simulink model "fault_detection_system_v3_updated"  (R2024a)
settings: Solver=FixedStepDiscrete  StartTime=0.0  StopTime=2.2  FixedStep=1e-4  RelTol=1e-3
settings Model: Creator=UJJWAL  LastModifiedBy=UJJWAL

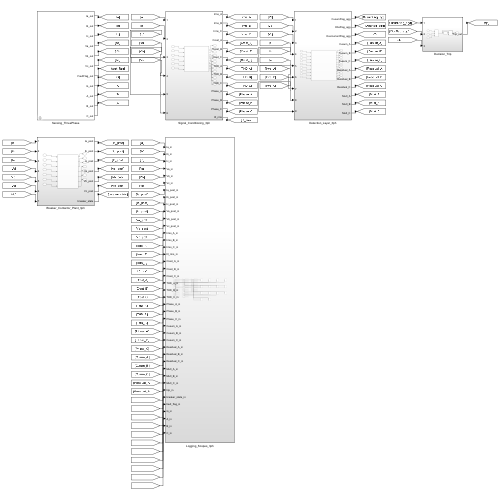
[thumbnail: Simulink's stored preview of the top-level diagram]
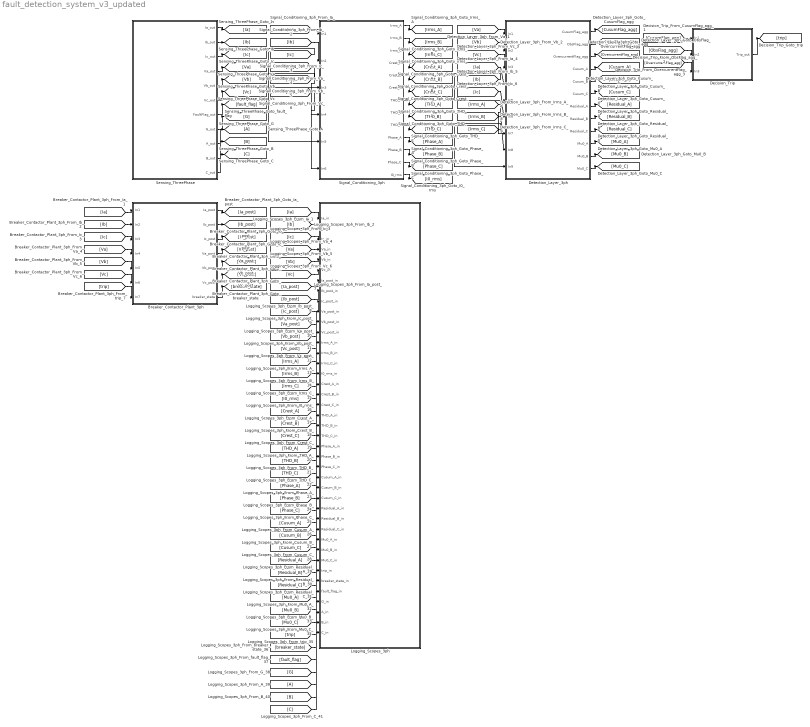
== system fault_detection_system_v3_updated ==
  Breaker_Contactor_Plant_3ph : Subsystem
  Decision_Trip : Subsystem
  Detection_Layer_3ph : Subsystem
  Logging_Scopes_3ph : Subsystem
  Logging_Scopes_3ph_From_A_39 : From
  Sensing_ThreePhase : Subsystem  mask{FaultG=off, FaultA=on, FaultB=on, FaultC=on, MechanismCode=6, Severity=1790.2024, RampDuration=0, FaultOnsetTime=0.7, FaultDuration=1, NoiseSeed=2700, NoiseI=0.3, NoiseV=3}
      mask prompts: FaultG "Ground involved (G)"; FaultA "Phase A involved"; FaultB "Phase B involved"; FaultC "Phase C involved"; MechanismCode "Mechanism code (1=Healthy, 2=ShortCircuit, 3=Overcurrent, 4=Overvoltage, 5=Undervoltage, 6=OpenCircuit)"; RampDuration "Ramp duration (s)"; FaultOnsetTime "Fault onset time (s)"; FaultDuration "Fault duration (s)"; NoiseSeed "Noise seed"; NoiseI "Current sensor noise (A, per sample)"; NoiseV "Voltage sensor noise (V, per sample)"
  Sensing_ThreePhase_Goto_A : Goto
  Signal_Conditioning_3ph : Subsystem
  wires:
  Sensing_ThreePhase/1(Ia_out) -> [Ia]
  Sensing_ThreePhase/2(Ib_out) -> [Ib]
  Sensing_ThreePhase/3(Ic_out) -> [Ic]
  Sensing_ThreePhase/4(Va_out) -> [Va]
  Sensing_ThreePhase/5(Vb_out) -> [Vb]
  Sensing_ThreePhase/6(Vc_out) -> [Vc]
  Sensing_ThreePhase/7(FaultFlag_out) -> [fault_flag]
  Sensing_ThreePhase/8(G_out) -> [G]
  Sensing_ThreePhase/9(A_out) -> Sensing_ThreePhase_Goto_A/1
  Sensing_ThreePhase/10(B_out) -> [B]
  Sensing_ThreePhase/11(C_out) -> [C]
  Signal_Conditioning_3ph/1(Irms_A) -> [Irms_A]
  Signal_Conditioning_3ph/2(Irms_B) -> [Irms_B]
  Signal_Conditioning_3ph/3(Irms_C) -> [Irms_C]
  Signal_Conditioning_3ph/4(Crest_A) -> [Crest_A]
  Signal_Conditioning_3ph/5(Crest_B) -> [Crest_B]
  Signal_Conditioning_3ph/6(Crest_C) -> [Crest_C]
  Signal_Conditioning_3ph/7(THD_A) -> [THD_A]
  Signal_Conditioning_3ph/8(THD_B) -> [THD_B]
  Signal_Conditioning_3ph/9(THD_C) -> [THD_C]
  Signal_Conditioning_3ph/10(Phase_A) -> [Phase_A]
  Signal_Conditioning_3ph/11(Phase_B) -> [Phase_B]
  Signal_Conditioning_3ph/12(Phase_C) -> [Phase_C]
  Signal_Conditioning_3ph/13(I0_rms) -> [I0_rms]
  Detection_Layer_3ph/1(CusumFlag_agg) -> [CusumFlag_agg]
  Detection_Layer_3ph/2(ObsFlag_agg) -> [ObsFlag_agg]
  Detection_Layer_3ph/3(OvercurrentFlag_agg) -> [OvercurrentFlag_agg]
  Detection_Layer_3ph/4(Cusum_A) -> [Cusum_A]
  Detection_Layer_3ph/5(Cusum_B) -> [Cusum_B]
  Detection_Layer_3ph/6(Cusum_C) -> [Cusum_C]
  Detection_Layer_3ph/7(Residual_A) -> [Residual_A]
  Detection_Layer_3ph/8(Residual_B) -> [Residual_B]
  Detection_Layer_3ph/9(Residual_C) -> [Residual_C]
  Detection_Layer_3ph/10(Mu0_A) -> [Mu0_A]
  Detection_Layer_3ph/11(Mu0_B) -> [Mu0_B]
  Detection_Layer_3ph/12(Mu0_C) -> [Mu0_C]
  Decision_Trip/1(Trip_out) -> [trip]
  Breaker_Contactor_Plant_3ph/1(Ia_post) -> [Ia_post]
  Breaker_Contactor_Plant_3ph/2(Ib_post) -> [Ib_post]
  Breaker_Contactor_Plant_3ph/3(Ic_post) -> [Ic_post]
  Breaker_Contactor_Plant_3ph/4(Va_post) -> [Va_post]
  Breaker_Contactor_Plant_3ph/5(Vb_post) -> [Vb_post]
  Breaker_Contactor_Plant_3ph/6(Vc_post) -> [Vc_post]
  Breaker_Contactor_Plant_3ph/7(breaker_state) -> [breaker_state]
  [Ia] -> Signal_Conditioning_3ph/1(In1)
  [Ib] -> Signal_Conditioning_3ph/2(In2)
  [Ic] -> Signal_Conditioning_3ph/3(In3)
  [Va] -> Signal_Conditioning_3ph/4(In4)
  [Vb] -> Signal_Conditioning_3ph/5(In5)
  [Vc] -> Signal_Conditioning_3ph/6(In6)
  [Va] -> Detection_Layer_3ph/1(In1)
  [Vb] -> Detection_Layer_3ph/2(In2)
  [Vc] -> Detection_Layer_3ph/3(In3)
  [Ia] -> Detection_Layer_3ph/4(In4)
  [Ib] -> Detection_Layer_3ph/5(In5)
  [Ic] -> Detection_Layer_3ph/6(In6)
  [Irms_A] -> Detection_Layer_3ph/7(In7)
  [Irms_B] -> Detection_Layer_3ph/8(In8)
  [Irms_C] -> Detection_Layer_3ph/9(In9)
  [CusumFlag_agg] -> Decision_Trip/1(In1)
  [ObsFlag_agg] -> Decision_Trip/2(In2)
  [OvercurrentFlag_agg] -> Decision_Trip/3(In3)
  [Ia] -> Breaker_Contactor_Plant_3ph/1(In1)
  [Ib] -> Breaker_Contactor_Plant_3ph/2(In2)
  [Ic] -> Breaker_Contactor_Plant_3ph/3(In3)
  [Va] -> Breaker_Contactor_Plant_3ph/4(In4)
  [Vb] -> Breaker_Contactor_Plant_3ph/5(In5)
  [Vc] -> Breaker_Contactor_Plant_3ph/6(In6)
  [trip] -> Breaker_Contactor_Plant_3ph/7(In7)
  [Ia] -> Logging_Scopes_3ph/1(Ia_in)
  [Ib] -> Logging_Scopes_3ph/2(Ib_in)
  [Ic] -> Logging_Scopes_3ph/3(Ic_in)
  [Va] -> Logging_Scopes_3ph/4(Va_in)
  [Vb] -> Logging_Scopes_3ph/5(Vb_in)
  [Vc] -> Logging_Scopes_3ph/6(Vc_in)
  [Ia_post] -> Logging_Scopes_3ph/7(Ia_post_in)
  [Ib_post] -> Logging_Scopes_3ph/8(Ib_post_in)
  [Ic_post] -> Logging_Scopes_3ph/9(Ic_post_in)
  [Va_post] -> Logging_Scopes_3ph/10(Va_post_in)
  [Vb_post] -> Logging_Scopes_3ph/11(Vb_post_in)
  [Vc_post] -> Logging_Scopes_3ph/12(Vc_post_in)
  [Irms_A] -> Logging_Scopes_3ph/13(Irms_A_in)
  [Irms_B] -> Logging_Scopes_3ph/14(Irms_B_in)
  [Irms_C] -> Logging_Scopes_3ph/15(Irms_C_in)
  [I0_rms] -> Logging_Scopes_3ph/16(I0_rms_in)
  [Crest_A] -> Logging_Scopes_3ph/17(Crest_A_in)
  [Crest_B] -> Logging_Scopes_3ph/18(Crest_B_in)
  [Crest_C] -> Logging_Scopes_3ph/19(Crest_C_in)
  [THD_A] -> Logging_Scopes_3ph/20(THD_A_in)
  [THD_B] -> Logging_Scopes_3ph/21(THD_B_in)
  [THD_C] -> Logging_Scopes_3ph/22(THD_C_in)
  [Phase_A] -> Logging_Scopes_3ph/23(Phase_A_in)
  [Phase_B] -> Logging_Scopes_3ph/24(Phase_B_in)
  [Phase_C] -> Logging_Scopes_3ph/25(Phase_C_in)
  [Cusum_A] -> Logging_Scopes_3ph/26(Cusum_A_in)
  [Cusum_B] -> Logging_Scopes_3ph/27(Cusum_B_in)
  [Cusum_C] -> Logging_Scopes_3ph/28(Cusum_C_in)
  [Residual_A] -> Logging_Scopes_3ph/29(Residual_A_in)
  [Residual_B] -> Logging_Scopes_3ph/30(Residual_B_in)
  [Residual_C] -> Logging_Scopes_3ph/31(Residual_C_in)
  [Mu0_A] -> Logging_Scopes_3ph/32(Mu0_A_in)
  [Mu0_B] -> Logging_Scopes_3ph/33(Mu0_B_in)
  [Mu0_C] -> Logging_Scopes_3ph/34(Mu0_C_in)
  [trip] -> Logging_Scopes_3ph/35(trip_in)
  [breaker_state] -> Logging_Scopes_3ph/36(breaker_state_in)
  [fault_flag] -> Logging_Scopes_3ph/37(fault_flag_in)
  [G] -> Logging_Scopes_3ph/38(G_in)
  Logging_Scopes_3ph_From_A_39/1 -> Logging_Scopes_3ph/39(A_in)
  [B] -> Logging_Scopes_3ph/40(B_in)
  [C] -> Logging_Scopes_3ph/41(C_in)

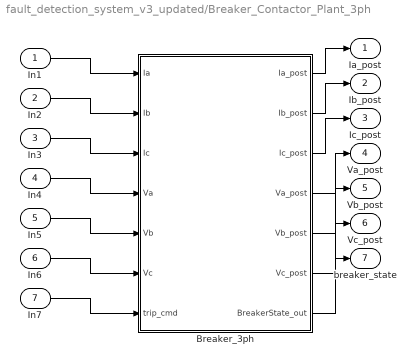
== system fault_detection_system_v3_updated/Breaker_Contactor_Plant_3ph ==
  In1 : Inport
  In2 : Inport  Port=2
  In3 : Inport  Port=3
  In4 : Inport  Port=4
  In5 : Inport  Port=5
  In6 : Inport  Port=6
  In7 : Inport  Port=7
  Breaker_3ph : MATLAB Function  TreatAsAtomicUnit=on
  Ia_post : Outport
  Ib_post : Outport  Port=2
  Ic_post : Outport  Port=3
  Va_post : Outport  Port=4
  Vb_post : Outport  Port=5
  Vc_post : Outport  Port=6
  breaker_state : Outport  Port=7
  wires:
  Breaker_3ph/1(Ia_post) -> Ia_post/1
  Breaker_3ph/2(Ib_post) -> Ib_post/1
  Breaker_3ph/3(Ic_post) -> Ic_post/1
  Breaker_3ph/4(Va_post) -> Va_post/1
  Breaker_3ph/5(Vb_post) -> Vb_post/1
  Breaker_3ph/6(Vc_post) -> Vc_post/1
  Breaker_3ph/7(BreakerState_out) -> breaker_state/1
  In1/1 -> Breaker_3ph/1(Ia)
  In2/1 -> Breaker_3ph/2(Ib)
  In3/1 -> Breaker_3ph/3(Ic)
  In4/1 -> Breaker_3ph/4(Va)
  In5/1 -> Breaker_3ph/5(Vb)
  In6/1 -> Breaker_3ph/6(Vc)
  In7/1 -> Breaker_3ph/7(trip_cmd)

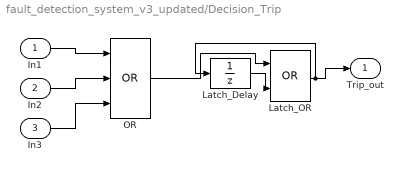
== system fault_detection_system_v3_updated/Decision_Trip ==
  In1 : Inport
  In2 : Inport  Port=2
  In3 : Inport  Port=3
  Latch_Delay : UnitDelay  SampleTime=-1  HasFrameUpgradeWarning=on
  Latch_OR : Logic  Operator=OR  AllPortsSameDT=off  OutDataTypeStr=boolean
  OR : Logic  Operator=OR  Inputs=3  AllPortsSameDT=off  OutDataTypeStr=boolean
  Trip_out : Outport
  wires:
  In1/1 -> OR/1
  In2/1 -> OR/2
  In3/1 -> OR/3
  OR/1 -> Latch_OR/1
  Latch_Delay/1 -> Latch_OR/2
  Latch_OR/1 -> Latch_Delay/1, Trip_out/1

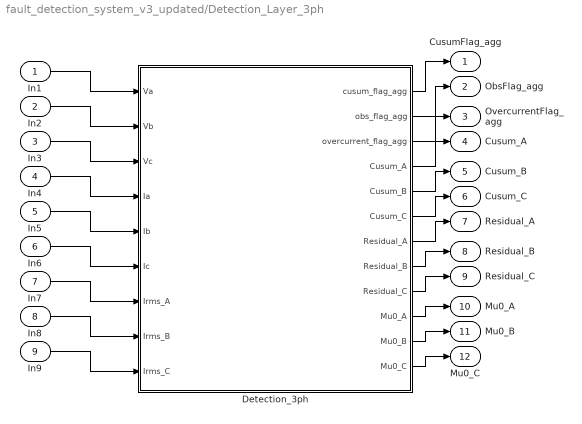
== system fault_detection_system_v3_updated/Detection_Layer_3ph ==
  In1 : Inport
  In2 : Inport  Port=2
  In3 : Inport  Port=3
  In4 : Inport  Port=4
  In5 : Inport  Port=5
  In6 : Inport  Port=6
  In7 : Inport  Port=7
  In8 : Inport  Port=8
  In9 : Inport  Port=9
  Detection_3ph : MATLAB Function  TreatAsAtomicUnit=on
  CusumFlag_agg : Outport
  ObsFlag_agg : Outport  Port=2
  OvercurrentFlag_agg : Outport  Port=3
  Cusum_A : Outport  Port=4
  Cusum_B : Outport  Port=5
  Cusum_C : Outport  Port=6
  Residual_A : Outport  Port=7
  Residual_B : Outport  Port=8
  Residual_C : Outport  Port=9
  Mu0_A : Outport  Port=10
  Mu0_B : Outport  Port=11
  Mu0_C : Outport  Port=12
  wires:
  Detection_3ph/1(cusum_flag_agg) -> CusumFlag_agg/1
  Detection_3ph/2(obs_flag_agg) -> ObsFlag_agg/1
  Detection_3ph/3(overcurrent_flag_agg) -> OvercurrentFlag_agg/1
  Detection_3ph/4(Cusum_A) -> Cusum_A/1
  Detection_3ph/5(Cusum_B) -> Cusum_B/1
  Detection_3ph/6(Cusum_C) -> Cusum_C/1
  Detection_3ph/7(Residual_A) -> Residual_A/1
  Detection_3ph/8(Residual_B) -> Residual_B/1
  Detection_3ph/9(Residual_C) -> Residual_C/1
  Detection_3ph/10(Mu0_A) -> Mu0_A/1
  Detection_3ph/11(Mu0_B) -> Mu0_B/1
  Detection_3ph/12(Mu0_C) -> Mu0_C/1
  In1/1 -> Detection_3ph/1(Va)
  In2/1 -> Detection_3ph/2(Vb)
  In3/1 -> Detection_3ph/3(Vc)
  In4/1 -> Detection_3ph/4(Ia)
  In5/1 -> Detection_3ph/5(Ib)
  In6/1 -> Detection_3ph/6(Ic)
  In7/1 -> Detection_3ph/7(Irms_A)
  In8/1 -> Detection_3ph/8(Irms_B)
  In9/1 -> Detection_3ph/9(Irms_C)

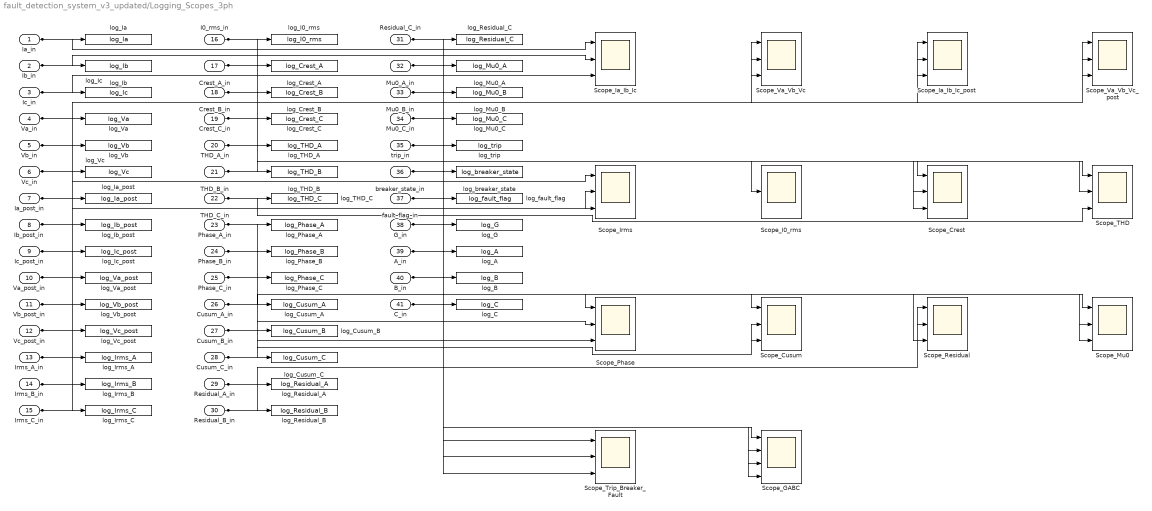
== system fault_detection_system_v3_updated/Logging_Scopes_3ph ==
  Ia_in : Inport
  Ib_in : Inport  Port=2
  Ic_in : Inport  Port=3
  Va_in : Inport  Port=4
  Vb_in : Inport  Port=5
  Vc_in : Inport  Port=6
  Ia_post_in : Inport  Port=7
  Ib_post_in : Inport  Port=8
  Ic_post_in : Inport  Port=9
  Va_post_in : Inport  Port=10
  Vb_post_in : Inport  Port=11
  Vc_post_in : Inport  Port=12
  Irms_A_in : Inport  Port=13
  Irms_B_in : Inport  Port=14
  Irms_C_in : Inport  Port=15
  I0_rms_in : Inport  Port=16
  Crest_A_in : Inport  Port=17
  Crest_B_in : Inport  Port=18
  Crest_C_in : Inport  Port=19
  THD_A_in : Inport  Port=20
  THD_B_in : Inport  Port=21
  THD_C_in : Inport  Port=22
  Phase_A_in : Inport  Port=23
  Phase_B_in : Inport  Port=24
  Phase_C_in : Inport  Port=25
  Cusum_A_in : Inport  Port=26
  Cusum_B_in : Inport  Port=27
  Cusum_C_in : Inport  Port=28
  Residual_A_in : Inport  Port=29
  Residual_B_in : Inport  Port=30
  Residual_C_in : Inport  Port=31
  Mu0_A_in : Inport  Port=32
  Mu0_B_in : Inport  Port=33
  Mu0_C_in : Inport  Port=34
  trip_in : Inport  Port=35
  breaker_state_in : Inport  Port=36
  fault_flag_in : Inport  Port=37
  G_in : Inport  Port=38
  A_in : Inport  Port=39
  B_in : Inport  Port=40
  C_in : Inport  Port=41
  Scope_Crest : Scope  NumInputPorts=3
  Scope_Cusum : Scope  NumInputPorts=3
  Scope_GABC : Scope  NumInputPorts=4
  Scope_I0_rms : Scope
  Scope_Ia_Ib_Ic : Scope  NumInputPorts=3
  Scope_Ia_Ib_Ic_post : Scope  NumInputPorts=3
  Scope_Irms : Scope  NumInputPorts=3
  Scope_Mu0 : Scope  NumInputPorts=3
  Scope_Phase : Scope  NumInputPorts=3
  Scope_Residual : Scope  NumInputPorts=3
  Scope_THD : Scope  NumInputPorts=3
  Scope_Trip_Breaker_Fault : Scope  NumInputPorts=3
  Scope_Va_Vb_Vc : Scope  NumInputPorts=3
  Scope_Va_Vb_Vc_post : Scope  NumInputPorts=3
  log_A : ToWorkspace  VariableName=log_A  SaveFormat=Timeseries  SampleTime=-1
  log_B : ToWorkspace  VariableName=log_B  SaveFormat=Timeseries  SampleTime=-1
  log_C : ToWorkspace  VariableName=log_C  SaveFormat=Timeseries  SampleTime=-1
  log_Crest_A : ToWorkspace  VariableName=log_Crest_A  SaveFormat=Timeseries  SampleTime=-1
  log_Crest_B : ToWorkspace  VariableName=log_Crest_B  SaveFormat=Timeseries  SampleTime=-1
  log_Crest_C : ToWorkspace  VariableName=log_Crest_C  SaveFormat=Timeseries  SampleTime=-1
  log_Cusum_A : ToWorkspace  VariableName=log_Cusum_A  SaveFormat=Timeseries  SampleTime=-1
  log_Cusum_B : ToWorkspace  VariableName=log_Cusum_B  SaveFormat=Timeseries  SampleTime=-1
  log_Cusum_C : ToWorkspace  VariableName=log_Cusum_C  SaveFormat=Timeseries  SampleTime=-1
  log_G : ToWorkspace  VariableName=log_G  SaveFormat=Timeseries  SampleTime=-1
  log_I0_rms : ToWorkspace  VariableName=log_I0_rms  SaveFormat=Timeseries  SampleTime=-1
  log_Ia : ToWorkspace  VariableName=log_Ia  SaveFormat=Timeseries  SampleTime=-1
  log_Ia_post : ToWorkspace  VariableName=log_Ia_post  SaveFormat=Timeseries  SampleTime=-1
  log_Ib : ToWorkspace  VariableName=log_Ib  SaveFormat=Timeseries  SampleTime=-1
  log_Ib_post : ToWorkspace  VariableName=log_Ib_post  SaveFormat=Timeseries  SampleTime=-1
  log_Ic : ToWorkspace  VariableName=log_Ic  SaveFormat=Timeseries  SampleTime=-1
  log_Ic_post : ToWorkspace  VariableName=log_Ic_post  SaveFormat=Timeseries  SampleTime=-1
  log_Irms_A : ToWorkspace  VariableName=log_Irms_A  SaveFormat=Timeseries  SampleTime=-1
  log_Irms_B : ToWorkspace  VariableName=log_Irms_B  SaveFormat=Timeseries  SampleTime=-1
  log_Irms_C : ToWorkspace  VariableName=log_Irms_C  SaveFormat=Timeseries  SampleTime=-1
  log_Mu0_A : ToWorkspace  VariableName=log_Mu0_A  SaveFormat=Timeseries  SampleTime=-1
  log_Mu0_B : ToWorkspace  VariableName=log_Mu0_B  SaveFormat=Timeseries  SampleTime=-1
  log_Mu0_C : ToWorkspace  VariableName=log_Mu0_C  SaveFormat=Timeseries  SampleTime=-1
  log_Phase_A : ToWorkspace  VariableName=log_Phase_A  SaveFormat=Timeseries  SampleTime=-1
  log_Phase_B : ToWorkspace  VariableName=log_Phase_B  SaveFormat=Timeseries  SampleTime=-1
  log_Phase_C : ToWorkspace  VariableName=log_Phase_C  SaveFormat=Timeseries  SampleTime=-1
  log_Residual_A : ToWorkspace  VariableName=log_Residual_A  SaveFormat=Timeseries  SampleTime=-1
  log_Residual_B : ToWorkspace  VariableName=log_Residual_B  SaveFormat=Timeseries  SampleTime=-1
  log_Residual_C : ToWorkspace  VariableName=log_Residual_C  SaveFormat=Timeseries  SampleTime=-1
  log_THD_A : ToWorkspace  VariableName=log_THD_A  SaveFormat=Timeseries  SampleTime=-1
  log_THD_B : ToWorkspace  VariableName=log_THD_B  SaveFormat=Timeseries  SampleTime=-1
  log_THD_C : ToWorkspace  VariableName=log_THD_C  SaveFormat=Timeseries  SampleTime=-1
  log_Va : ToWorkspace  VariableName=log_Va  SaveFormat=Timeseries  SampleTime=-1
  log_Va_post : ToWorkspace  VariableName=log_Va_post  SaveFormat=Timeseries  SampleTime=-1
  log_Vb : ToWorkspace  VariableName=log_Vb  SaveFormat=Timeseries  SampleTime=-1
  log_Vb_post : ToWorkspace  VariableName=log_Vb_post  SaveFormat=Timeseries  SampleTime=-1
  log_Vc : ToWorkspace  VariableName=log_Vc  SaveFormat=Timeseries  SampleTime=-1
  log_Vc_post : ToWorkspace  VariableName=log_Vc_post  SaveFormat=Timeseries  SampleTime=-1
  log_breaker_state : ToWorkspace  VariableName=log_breaker_state  SaveFormat=Timeseries  SampleTime=-1
  log_fault_flag : ToWorkspace  VariableName=log_fault_flag  SaveFormat=Timeseries  SampleTime=-1
  log_trip : ToWorkspace  VariableName=log_trip  SaveFormat=Timeseries  SampleTime=-1
  wires:
  Ia_in/1 -> log_Ia/1, Scope_Ia_Ib_Ic/1
  Ib_in/1 -> log_Ib/1, Scope_Ia_Ib_Ic/2
  Ic_in/1 -> log_Ic/1, Scope_Ia_Ib_Ic/3
  Va_in/1 -> log_Va/1, Scope_Va_Vb_Vc/1
  Vb_in/1 -> log_Vb/1, Scope_Va_Vb_Vc/2
  Vc_in/1 -> log_Vc/1, Scope_Va_Vb_Vc/3
  Ia_post_in/1 -> log_Ia_post/1, Scope_Ia_Ib_Ic_post/1
  Ib_post_in/1 -> log_Ib_post/1, Scope_Ia_Ib_Ic_post/2
  Ic_post_in/1 -> log_Ic_post/1, Scope_Ia_Ib_Ic_post/3
  Va_post_in/1 -> log_Va_post/1, Scope_Va_Vb_Vc_post/1
  Vb_post_in/1 -> log_Vb_post/1, Scope_Va_Vb_Vc_post/2
  Vc_post_in/1 -> log_Vc_post/1, Scope_Va_Vb_Vc_post/3
  Irms_A_in/1 -> log_Irms_A/1, Scope_Irms/1
  Irms_B_in/1 -> log_Irms_B/1, Scope_Irms/2
  Irms_C_in/1 -> log_Irms_C/1, Scope_Irms/3
  I0_rms_in/1 -> log_I0_rms/1, Scope_I0_rms/1
  Crest_A_in/1 -> log_Crest_A/1, Scope_Crest/1
  Crest_B_in/1 -> log_Crest_B/1, Scope_Crest/2
  Crest_C_in/1 -> log_Crest_C/1, Scope_Crest/3
  THD_A_in/1 -> log_THD_A/1, Scope_THD/1
  THD_B_in/1 -> log_THD_B/1, Scope_THD/2
  THD_C_in/1 -> log_THD_C/1, Scope_THD/3
  Phase_A_in/1 -> log_Phase_A/1, Scope_Phase/1
  Phase_B_in/1 -> log_Phase_B/1, Scope_Phase/2
  Phase_C_in/1 -> log_Phase_C/1, Scope_Phase/3
  Cusum_A_in/1 -> log_Cusum_A/1, Scope_Cusum/1
  Cusum_B_in/1 -> log_Cusum_B/1, Scope_Cusum/2
  Cusum_C_in/1 -> log_Cusum_C/1, Scope_Cusum/3
  Residual_A_in/1 -> log_Residual_A/1, Scope_Residual/1
  Residual_B_in/1 -> log_Residual_B/1, Scope_Residual/2
  Residual_C_in/1 -> log_Residual_C/1, Scope_Residual/3
  Mu0_A_in/1 -> log_Mu0_A/1, Scope_Mu0/1
  Mu0_B_in/1 -> log_Mu0_B/1, Scope_Mu0/2
  Mu0_C_in/1 -> log_Mu0_C/1, Scope_Mu0/3
  trip_in/1 -> log_trip/1, Scope_Trip_Breaker_Fault/1
  breaker_state_in/1 -> log_breaker_state/1, Scope_Trip_Breaker_Fault/2
  fault_flag_in/1 -> log_fault_flag/1, Scope_Trip_Breaker_Fault/3
  G_in/1 -> log_G/1, Scope_GABC/1
  A_in/1 -> log_A/1, Scope_GABC/2
  B_in/1 -> log_B/1, Scope_GABC/3
  C_in/1 -> log_C/1, Scope_GABC/4

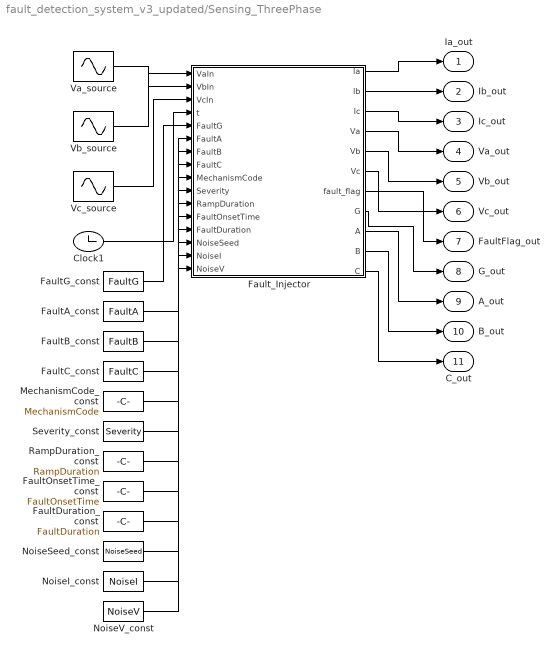
== system fault_detection_system_v3_updated/Sensing_ThreePhase ==
  Clock1 : Clock
  FaultA_const : Constant  Value=FaultA
  FaultB_const : Constant  Value=FaultB
  FaultC_const : Constant  Value=FaultC
  FaultDuration_const : Constant  Value=FaultDuration
  FaultG_const : Constant  Value=FaultG
  FaultOnsetTime_const : Constant  Value=FaultOnsetTime
  Fault_Injector : MATLAB Function  TreatAsAtomicUnit=on
  MechanismCode_const : Constant  Value=MechanismCode
  NoiseI_const : Constant  Value=NoiseI
  NoiseSeed_const : Constant  Value=NoiseSeed
  NoiseV_const : Constant  Value=NoiseV
  RampDuration_const : Constant  Value=RampDuration
  Severity_const : Constant  Value=Severity
  Va_source : Sin  Amplitude=325  Frequency=314.159  SampleTime=0
  Vb_source : Sin  Amplitude=325  Frequency=314.159  Phase=-2.0944  SampleTime=0
  Vc_source : Sin  Amplitude=325  Frequency=314.159  Phase=2.0944  SampleTime=0
  Ia_out : Outport
  Ib_out : Outport  Port=2
  Ic_out : Outport  Port=3
  Va_out : Outport  Port=4
  Vb_out : Outport  Port=5
  Vc_out : Outport  Port=6
  FaultFlag_out : Outport  Port=7
  G_out : Outport  Port=8
  A_out : Outport  Port=9
  B_out : Outport  Port=10
  C_out : Outport  Port=11
  wires:
  FaultG_const/1 -> Fault_Injector/5(FaultG)
  FaultA_const/1 -> Fault_Injector/6(FaultA)
  FaultB_const/1 -> Fault_Injector/7(FaultB)
  FaultC_const/1 -> Fault_Injector/8(FaultC)
  MechanismCode_const/1 -> Fault_Injector/9(MechanismCode)
  Severity_const/1 -> Fault_Injector/10(Severity)
  RampDuration_const/1 -> Fault_Injector/11(RampDuration)
  FaultOnsetTime_const/1 -> Fault_Injector/12(FaultOnsetTime)
  FaultDuration_const/1 -> Fault_Injector/13(FaultDuration)
  NoiseSeed_const/1 -> Fault_Injector/14(NoiseSeed)
  NoiseI_const/1 -> Fault_Injector/15(NoiseI)
  NoiseV_const/1 -> Fault_Injector/16(NoiseV)
  Va_source/1 -> Fault_Injector/1(VaIn)
  Vb_source/1 -> Fault_Injector/2(VbIn)
  Vc_source/1 -> Fault_Injector/3(VcIn)
  Clock1/1 -> Fault_Injector/4(t)
  Fault_Injector/1(Ia) -> Ia_out/1
  Fault_Injector/2(Ib) -> Ib_out/1
  Fault_Injector/3(Ic) -> Ic_out/1
  Fault_Injector/4(Va) -> Va_out/1
  Fault_Injector/5(Vb) -> Vb_out/1
  Fault_Injector/6(Vc) -> Vc_out/1
  Fault_Injector/7(fault_flag) -> FaultFlag_out/1
  Fault_Injector/8(G) -> G_out/1
  Fault_Injector/9(A) -> A_out/1
  Fault_Injector/10(B) -> B_out/1
  Fault_Injector/11(C) -> C_out/1

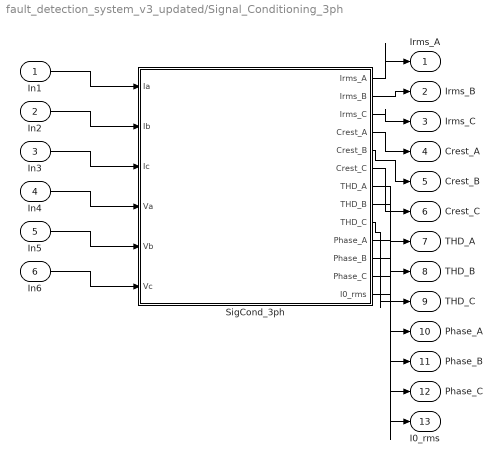
== system fault_detection_system_v3_updated/Signal_Conditioning_3ph ==
  In1 : Inport
  In2 : Inport  Port=2
  In3 : Inport  Port=3
  In4 : Inport  Port=4
  In5 : Inport  Port=5
  In6 : Inport  Port=6
  SigCond_3ph : MATLAB Function  TreatAsAtomicUnit=on
  Irms_A : Outport
  Irms_B : Outport  Port=2
  Irms_C : Outport  Port=3
  Crest_A : Outport  Port=4
  Crest_B : Outport  Port=5
  Crest_C : Outport  Port=6
  THD_A : Outport  Port=7
  THD_B : Outport  Port=8
  THD_C : Outport  Port=9
  Phase_A : Outport  Port=10
  Phase_B : Outport  Port=11
  Phase_C : Outport  Port=12
  I0_rms : Outport  Port=13
  wires:
  SigCond_3ph/1(Irms_A) -> Irms_A/1
  SigCond_3ph/2(Irms_B) -> Irms_B/1
  SigCond_3ph/3(Irms_C) -> Irms_C/1
  SigCond_3ph/4(Crest_A) -> Crest_A/1
  SigCond_3ph/5(Crest_B) -> Crest_B/1
  SigCond_3ph/6(Crest_C) -> Crest_C/1
  SigCond_3ph/7(THD_A) -> THD_A/1
  SigCond_3ph/8(THD_B) -> THD_B/1
  SigCond_3ph/9(THD_C) -> THD_C/1
  SigCond_3ph/10(Phase_A) -> Phase_A/1
  SigCond_3ph/11(Phase_B) -> Phase_B/1
  SigCond_3ph/12(Phase_C) -> Phase_C/1
  SigCond_3ph/13(I0_rms) -> I0_rms/1
  In1/1 -> SigCond_3ph/1(Ia)
  In2/1 -> SigCond_3ph/2(Ib)
  In3/1 -> SigCond_3ph/3(Ic)
  In4/1 -> SigCond_3ph/4(Va)
  In5/1 -> SigCond_3ph/5(Vb)
  In6/1 -> SigCond_3ph/6(Vc)

== matlab function fault_detection_system_v3_updated/Breaker_Contactor_Plant_3ph/Breaker_3ph ==
  data: Ia input; Ia_post output; Ib input; Ic input; Va input; Vb input; Vc input; trip_cmd input; Ib_post output; Ic_post output; Va_post output; Vb_post output; Vc_post output; BreakerState_out output
function [Ia_post,Ib_post,Ic_post,Va_post,Vb_post,Vc_post,BreakerState_out] = breaker_3ph(Ia,Ib,Ic,Va,Vb,Vc,trip_cmd)
%#codegen
% Gang-operated 3-pole breaker: trip opens ALL three phases together
persistent state
if isempty(state), state = 0; end
state = max(state, double(trip_cmd));
Ia_post = Ia * (1 - state); Ib_post = Ib * (1 - state); Ic_post = Ic * (1 - state);
Va_post = Va * (1 - state); Vb_post = Vb * (1 - state); Vc_post = Vc * (1 - state);
BreakerState_out = state;

== matlab function fault_detection_system_v3_updated/Signal_Conditioning_3ph/SigCond_3ph ==
  data: Ia input; Irms_A output; Ib input; Ic input; Va input; Vb input; Vc input; Irms_B output; Irms_C output; Crest_A output; Crest_B output; Crest_C output; THD_A output; THD_B output; THD_C output; Phase_A output; Phase_B output; Phase_C output; I0_rms output
function [Irms_A,Irms_B,Irms_C,Crest_A,Crest_B,Crest_C,THD_A,THD_B,THD_C,Phase_A,Phase_B,Phase_C,I0_rms] = sigcond_3ph(Ia,Ib,Ic,Va,Vb,Vc)
%#codegen
persistent bufI bufV bufI0 idx N
if isempty(idx)
    N = 200; bufI = zeros(3,N); bufV = zeros(3,N); bufI0 = zeros(1,N); idx = 1;
end

% Sensor noise is already in the inputs (added in Fault_Injector)
I = [Ia, Ib, Ic];
V = [Va, Vb, Vc];

I0 = (I(1) + I(2) + I(3)) / 3;

bufI(:,idx) = I; bufV(:,idx) = V; bufI0(idx) = I0; idx = mod(idx, N) + 1;
Irms = sqrt(mean(bufI.^2, 2));
I0_rms = sqrt(mean(bufI0.^2));
Crest = max(abs(bufI), [], 2) ./ max(Irms, 1e-6);
THD = zeros(3,1); Phase = zeros(3,1);
for p = 1:3
    Fi = fft(bufI(p,:)); Fv = fft(bufV(p,:));
    fundBin = round(50 * N / 1e4) + 1;
    fundMag = abs(Fi(fundBin));
    harmMag = sqrt(sum(abs(Fi(fundBin+1:round(N/2))).^2));
    THD(p) = harmMag / max(fundMag, 1e-6);
    Phase(p) = angle(Fv(fundBin)) - angle(Fi(fundBin));
end
Irms_A=Irms(1); Irms_B=Irms(2); Irms_C=Irms(3);
Crest_A=Crest(1); Crest_B=Crest(2); Crest_C=Crest(3);
THD_A=THD(1); THD_B=THD(2); THD_C=THD(3);
Phase_A=Phase(1); Phase_B=Phase(2); Phase_C=Phase(3);

== matlab function fault_detection_system_v3_updated/Sensing_ThreePhase/Fault_Injector ==
  data: VaIn input; Ia output; VbIn input; VcIn input; t input; FaultG input; FaultA input; FaultB input; FaultC input; MechanismCode input; Severity input; RampDuration input; FaultOnsetTime input; FaultDuration input; NoiseSeed input; NoiseI input; NoiseV input; Ib output; Ic output; Va output; Vb output; Vc output; fault_flag output; G output; A output; B output; C output
%% fault_injection_core.m
%
% SINGLE SOURCE for the Fault_Injector block. model_code_v3_updated.m reads
% this file with fileread() and pastes it into the MATLAB Function block, so
% the block and this file cannot drift apart. Edit the physics here only.
% It can also be called standalone for unit tests; run `clear
% fault_injection_core` between runs because it keeps persistent state.
%
% PHYSICS
%   Each phase is a series inductance L feeding a node. The node has the
%   load conductance Y_load (1/5 Ohm per phase) plus a fault admittance
%   Y_f. The fault is a star network: every involved phase connects through
%   its own fault resistance (= Severity) to a common star point, and that
%   star point connects to ground through the grounding resistor R_NGR
%   when G = 1. Eliminating the star point (Kron reduction) gives
%       Y_f = diag(g) - g*g'/(sum(g) + g_ground)
%   so the ground path is in SERIES with the fault resistance, not in
%   parallel. LL has no ground return (I0 = 0). LLG, LG and LLLG do
%   (I0 ~= 0 unless the sources are balanced across all three phases,
%   which is why LLL and LLLG look identical).
%   Node voltage = inv(Y_total)*I, source = L*dI/dt + node voltage, solved
%   with backward Euler, so it is stable for any severity.
%
% MECHANISMS (MechanismCode)
%   1 Healthy | 2 ShortCircuit (Severity = fault R, Ohm)
%   3 Overcurrent (Severity = new load R, Ohm)
%   4 Overvoltage / 5 Undervoltage (Severity = source scale factor)
%   6 OpenCircuit (Severity = new load R, Ohm, >= 500)
%
% SENSOR NOISE
%   Gaussian noise (NoiseI amps, NoiseV volts, per sample) is added to the
%   OUTPUTS only. The internal current state stays clean, so the noise
%   models a sensor, and every logged channel (including the raw Ia/Va
%   samples the extractor uses) sees it. NoiseSeed seeds a private
%   xorshift32 generator, so a given seed reproduces the same noise.
%   Terminology: LG/LL/LLG are unsymmetrical faults; only LLL/LLLG are
%   symmetrical. All five are grouped as the ShortCircuit mechanism.
function [Ia,Ib,Ic,Va,Vb,Vc,fault_flag,G,A,B,C] = fault_injection_core(VaIn,VbIn,VcIn,t,FaultG,FaultA,FaultB,FaultC,MechanismCode,Severity,RampDuration,FaultOnsetTime,FaultDuration,NoiseSeed,NoiseI,NoiseV)
%#codegen
persistent I_s faultSamples rngState initialized
if isempty(initialized)
    I_s = zeros(3,1); faultSamples = 0; initialized = true;
    s0 = mod(double(NoiseSeed) * 2654435761 + 2463534242, 4294967296);
    if s0 == 0
        s0 = 1;
    end
    rngState = uint32(s0);
    for w = 1:8   % warm-up so small seeds do not give correlated first draws
        rngState = bitxor(rngState, bitshift(rngState, 13));
        rngState = bitxor(rngState, bitshift(rngState, -17));
        rngState = bitxor(rngState, bitshift(rngState, 5));
    end
end

Ts = 1e-4;        % must match the model FixedStep
L = 0.02;         % H per phase
R_normal = 5;     % Ohm, healthy load
R_NGR = 0.5;      % Ohm, neutral grounding resistor (ground return path)

fault_active = (t >= FaultOnsetTime) && (t < FaultOnsetTime + FaultDuration);
if fault_active
    faultSamples = faultSamples + 1;
else
    faultSamples = 0;
end
rampSamples = max(1, round(RampDuration / Ts));
frac = min(1, faultSamples / rampSamples);   % RampDuration = 0 -> full effect at once

flags = [FaultA; FaultB; FaultC];
V_in = [VaIn; VbIn; VcIn];
V_eff = V_in;
Y_load = diag([1/R_normal, 1/R_normal, 1/R_normal]);
Y_f = zeros(3,3);

if fault_active
    if MechanismCode == 2 % ShortCircuit
        g_f = 1 / Severity;
        g_g = (FaultG > 0.5) * (1 / R_NGR);
        g_vec = flags * g_f * frac;
        g_sum = sum(g_vec) + g_g;
        if g_sum > 0
            for i = 1:3
                for j = 1:3
                    if i == j
                        Y_f(i,j) = g_vec(i) - (g_vec(i)^2)/g_sum;
                    else
                        Y_f(i,j) = - (g_vec(i)*g_vec(j))/g_sum;
                    end
                end
            end
        end
    elseif MechanismCode == 3 % Overcurrent
        for i = 1:3
            if flags(i) > 0.5
                Y_load(i,i) = 1 / (R_normal + frac*(Severity - R_normal));
            end
        end
    elseif MechanismCode == 4 || MechanismCode == 5 % Over/Undervoltage
        for i = 1:3
            if flags(i) > 0.5
                V_eff(i) = V_in(i) * (1 + frac*(Severity - 1));
            end
        end
    elseif MechanismCode == 6 % OpenCircuit
        for i = 1:3
            if flags(i) > 0.5
                R_eff = R_normal + frac*(Severity - R_normal);
                Y_load(i,i) = 1 / R_eff;
            end
        end
    end
end

Y_total = Y_load + Y_f;
Z = inv(Y_total);
I_next = ( (L/Ts)*eye(3) + Z ) \ ( (L/Ts)*I_s + V_eff );
I_s = I_next;

% Sensor noise: 6 independent N(0,1) draws (Box-Muller on xorshift32)
n6 = zeros(6,1);
for k = 1:6
    u = zeros(2,1);
    for m = 1:2
        rngState = bitxor(rngState, bitshift(rngState, 13));
        rngState = bitxor(rngState, bitshift(rngState, -17));
        rngState = bitxor(rngState, bitshift(rngState, 5));
        u(m) = (double(rngState) + 0.5) / 4294967296;
    end
    n6(k) = sqrt(-2*log(u(1))) * cos(2*pi*u(2));
end

Ia = I_s(1) + NoiseI*n6(1); Ib = I_s(2) + NoiseI*n6(2); Ic = I_s(3) + NoiseI*n6(3);
Va = V_eff(1) + NoiseV*n6(4); Vb = V_eff(2) + NoiseV*n6(5); Vc = V_eff(3) + NoiseV*n6(6);
fault_flag = fault_active;
G = double(FaultG); A = double(FaultA); B = double(FaultB); C = double(FaultC);
end

== matlab function fault_detection_system_v3_updated/Detection_Layer_3ph/Detection_3ph ==
  data: Va input; cusum_flag_agg output; Vb input; Vc input; Ia input; Ib input; Ic input; Irms_A input; Irms_B input; Irms_C input; obs_flag_agg output; overcurrent_flag_agg output; Cusum_A output; Cusum_B output; Cusum_C output; Residual_A output; Residual_B output; Residual_C output; Mu0_A output; Mu0_B output; Mu0_C output
function [cusum_flag_agg,obs_flag_agg,overcurrent_flag_agg,Cusum_A,Cusum_B,Cusum_C,Residual_A,Residual_B,Residual_C,Mu0_A,Mu0_B,Mu0_C] = detection_3ph(Va,Vb,Vc,Ia,Ib,Ic,Irms_A,Irms_B,Irms_C)
    persistent mu0 var0 g_pos g_neg initialized sampleCount WARMUP_SAMPLES SETTLE_SAMPLES settleCount

    if isempty(initialized)
        mu0 = zeros(3,1);
        var0 = ones(3,1) * 0.01; % Initialize with small variance
        g_pos = zeros(3,1);
        g_neg = zeros(3,1);
        initialized = true;
        sampleCount = 0;
        WARMUP_SAMPLES = 500;
        SETTLE_SAMPLES = 400;
        settleCount = 0;
    end

    sampleCount = sampleCount + 1;

    Irms = [Irms_A; Irms_B; Irms_C];
    err = Irms - mu0;
    residual = abs(err);

    % MINIMUM NOISE FLOOR CLAMP
    % Prevents the learning standard deviation from dropping to zero
    MIN_NOISE_FLOOR = 0.05;
    std0 = max(sqrt(var0), MIN_NOISE_FLOOR);

    % Adaptive detection thresholds
    k = 1.0 * std0; % Adaptive CUSUM drift/slack
    H_THRESH = 10 * std0; % Adaptive CUSUM trip threshold
    OVERCURRENT_THRESH = mu0 + 15 * std0; % Adaptive overcurrent limit

    if sampleCount <= WARMUP_SAMPLES
        if sampleCount > SETTLE_SAMPLES
            settleCount = settleCount + 1;
            delta = Irms - mu0;
            mu0 = mu0 + delta / settleCount;
            var0 = var0 + (delta .* (Irms - mu0) - var0) / settleCount;
        end
        g_pos = zeros(3,1);
        g_neg = zeros(3,1);
        cusum_stat = zeros(3,1);
        cusum_flag_ph = false(3,1);
        obs_flag_ph = false(3,1);
        overcurrent_flag_ph = false(3,1);
    else
        g_pos = max(0, g_pos + err - k);
        g_neg = max(0, g_neg - err - k);

        cusum_stat = max(g_pos, g_neg);
        cusum_flag_ph = cusum_stat > H_THRESH;
        obs_flag_ph = residual > 5 * std0; % Adaptive residual bound
        overcurrent_flag_ph = Irms > OVERCURRENT_THRESH;

        % Freeze baseline tracking on any phase that exhibits a fault
        normal_mask = ~(cusum_flag_ph | obs_flag_ph | overcurrent_flag_ph);
        delta_norm = Irms(normal_mask) - mu0(normal_mask);
        mu0(normal_mask) = 0.999 * mu0(normal_mask) + 0.001 * Irms(normal_mask);
        var0(normal_mask) = 0.999 * var0(normal_mask) + 0.001 * (delta_norm.^2);
    end

    cusum_flag_agg = any(cusum_flag_ph);
    obs_flag_agg = any(obs_flag_ph);
    overcurrent_flag_agg = any(overcurrent_flag_ph);

    Cusum_A = cusum_stat(1); Cusum_B = cusum_stat(2); Cusum_C = cusum_stat(3);
    Residual_A = residual(1); Residual_B = residual(2); Residual_C = residual(3);
    Mu0_A = mu0(1); Mu0_B = mu0(2); Mu0_C = mu0(3);
end
